simulink model "sf_clutch"  (R2025b)
settings: Solver=ode45  StartTime=0.0  StopTime=10  RelTol=1e-6  AbsTol=1e-7
model workspace (MATLAB code in the model file):
  | % Load initial conditions and other information
  | 
  | load sf_clutch_data.mat;
undefined symbols (not defined in the file or in its folder): be, bv, Ie, Iv, muk, mus, R
Description:
  | Building a Clutch Lock-Up Model
  | 
  | This example shows how to use Simulink(R) to model and simulate a
  | rotating clutch system. Although modeling a clutch system is difficult
  | because of topological changes in the system dynamics during lockup, this
  | example shows how Simulinks enabled subsystems feature easily handles
  | such problems. We illustrate how to employ important Simulink modeling
  | concepts in the creation of the clutch simulation. Designers can apply
  | these concepts to many models with strong discontinuities and constraints
  | that may change dynamically.
  | 
  | In the example, we use enabled subsystems to build the clutch
  | model. Two enabled subsystems model the clutch dynamics in either the
  | locked or unlocked position. After running the simulation, a GUI opens.
  | Checking any of the boxes on the GUI produces a plot of any of the
  | selected variables (versus time).
settings Model: ExtModeTrigMode=oneshot  ExtModeArmWhenConnect=off  ExtModeAutoUpdateStatusClock=off  Creator=The MathWorks, Inc.  LastModifiedBy=The MathWorks, Inc.
settings SolverCC: AutoScaleAbsTol=off  ZeroCrossAlgorithm=Adaptive  AlgebraicLoopSolver=TrustRegion  MaxZcPerStep=1.0
settings DataIOCC: ExternalInput=[]  InitialState=[]  SaveFormat=Array  SaveState=on  DSMLogging=off  ReturnWorkspaceOutputs=off  StateSaveName=x  TimeSaveName=t  OutputSaveName=y  SignalLoggingName=sf_clutch_signals
settings OptimizationCC: BlockReduction=off  ReuseModelBlockBuffer=off  ExpressionDepthLimit=2147483647.0  InitFltsAndDblsToZero=on  LifeSpan=inf  BufferReusableBoundary=off
settings DebuggingCC: SaveWithParameterizedLinksMsg=none  SignalResolutionControl=TryResolveAllWithWarning  MultiTaskDSMMsg=warning  MultiTaskCondExecSysMsg=none  SigSpecEnsureSampleTimeMsg=none  IntegerOverflowMsg=none  FcnCallInpInsideContextMsg=warning  UnconnectedInputMsg=warning  UnconnectedOutputMsg=warning  UnconnectedLineMsg=warning  BusObjectLabelMismatch=none  AllowSymbolicDim=off  StateNameClashWarn=warning  SFUnexpectedBacktrackingDiag=warning  SFNoUnconditionalDefaultTransitionDiag=warning  SFExecutionAtInitializationDiag=none  IntegerSaturationMsg=none  ArithmeticOperatorsInVariantConditions=warning
settings HardwareCC: ProdBitPerPointer=32.0  ProdBitPerSizeT=32.0  ProdBitPerPtrDiffT=32.0  ProdLargestAtomicFloat=None  ProdIntDivRoundTo=Undefined  ProdEndianess=Unspecified  ProdWordSize=32.0  ProdHWDeviceType=32-bit Generic
settings ModelReferenceCC: EnableRefExpFcnMdlSchedulingChecks=on  PropagateSignalLabelsOutOfModel=off
settings SFSimCC: SimUseLocalCustomCode=off  CustomCodeUndefinedFunction=UseInterfaceOnly
settings RTWCC: RTWUseLocalCustomCode=off  GPUComputeCapability=3.5  DLArmComputeVersion=19.05
settings CodeAppCC: StateflowObjectComments=on
settings GRTTargetCC: TargetFcnLib=ansi_tfl_tmw.mat  TargetLangStandard=C89/C90 (ANSI)  CombineOutputUpdateFcns=off  GRTInterface=on
settings ConfigComp: CovMetricSettings=d  CovSaveCumulativeToWorkspaceVar=on  CovSaveSingleToWorkspaceVar=on  CovExternalEMLEnable=off

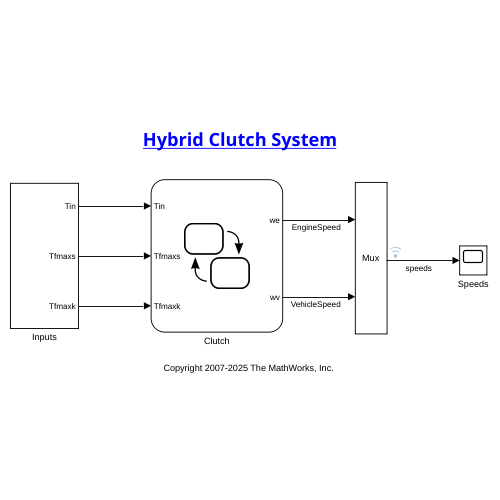
[thumbnail: Simulink's stored preview of the top-level diagram]
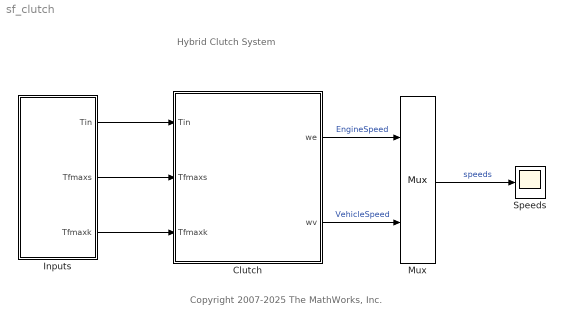
== system sf_clutch ==
  note: Copyright 2007-2025 The MathWorks, Inc.
  note: Hybrid Clutch System
  Clutch : Stateflow chart  TreatAsAtomicUnit=on
  Inputs : Subsystem
  Mux : Mux  Inputs=2
  Speeds : Scope
      settings: TimeSpan=10  ActiveDisplayYMinimum=-0.08933  ActiveDisplayYMaximum=0.80399
  wires:
  Clutch/1(we) -> Mux/1  "EngineSpeed"
  Clutch/2(wv) -> Mux/2  "VehicleSpeed"
  Mux/1 -> Speeds/1  "speeds"
  Inputs/1(Tin) -> Clutch/1(Tin)
  Inputs/2(Tfmaxs) -> Clutch/2(Tfmaxs)
  Inputs/3(Tfmaxk) -> Clutch/3(Tfmaxk)

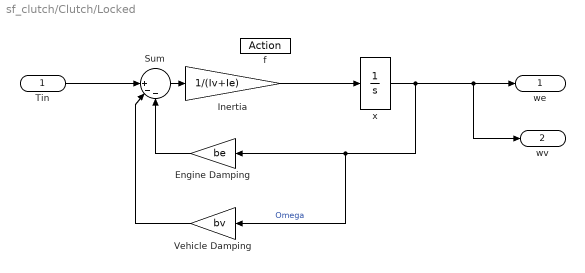
== system sf_clutch/Clutch/Locked ==
  Tin : Inport
  f : ActionPort
      settings: CopyFcn=Stateflow.SLINSF.SimulinkMan.removeBlockPreDeleteFcn  PreDeleteFcn=Stateflow.SLINSF.SimulinkMan.unsafePredeleteFcn
  Engine Damping : Gain  Gain=be  SaturateOnIntegerOverflow=on  OutDataTypeStr=Inherit: Same as input  ParamDataTypeStr=Inherit: Same as input
  Inertia : Gain  Gain=1/(Iv+Ie)  SaturateOnIntegerOverflow=on  OutDataTypeStr=Inherit: Same as input  ParamDataTypeStr=Inherit: Same as input
  Sum : Sum  Inputs=||+--  InputSameDT=on  SaturateOnIntegerOverflow=on  OutDataTypeStr=Inherit: Same as first input
  Vehicle Damping : Gain  Gain=bv  SaturateOnIntegerOverflow=on  OutDataTypeStr=Inherit: Same as input  ParamDataTypeStr=Inherit: Same as input
  x : Integrator  ContinuousStateAttributes='w'
  we : Outport  VectorParamsAs1DForOutWhenUnconnected=off
  wv : Outport  Port=2  VectorParamsAs1DForOutWhenUnconnected=off
  wires:
  Sum/1 -> Inertia/1
  Tin/1 -> Sum/1
  x/1 -> wv/1, we/1, Engine Damping/1, Vehicle Damping/1  "Omega"
  Engine Damping/1 -> Sum/3
  Inertia/1 -> x/1
  Vehicle Damping/1 -> Sum/2

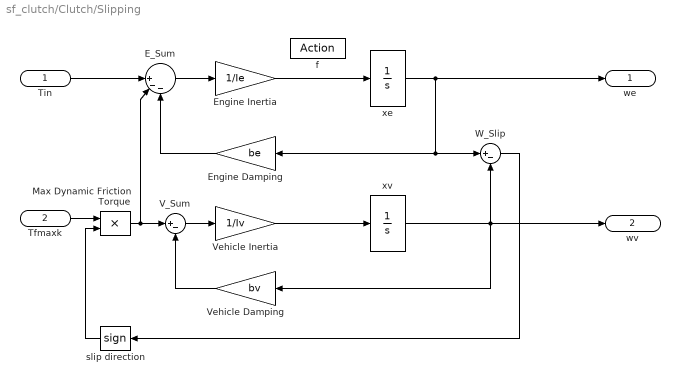
== system sf_clutch/Clutch/Slipping ==
  Tin : Inport
  Tfmaxk : Inport  Port=2
  f : ActionPort
      settings: CopyFcn=Stateflow.SLINSF.SimulinkMan.removeBlockPreDeleteFcn  PreDeleteFcn=Stateflow.SLINSF.SimulinkMan.unsafePredeleteFcn
  E_Sum : Sum  Inputs=||+--  InputSameDT=on  SaturateOnIntegerOverflow=on  OutDataTypeStr=Inherit: Same as first input
  Engine Damping : Gain  Gain=be  SaturateOnIntegerOverflow=on  OutDataTypeStr=Inherit: Same as input  ParamDataTypeStr=Inherit: Same as input
  Engine Inertia : Gain  Gain=1/Ie  SaturateOnIntegerOverflow=on  OutDataTypeStr=Inherit: Same as input  ParamDataTypeStr=Inherit: Same as input
  Max Dynamic Friction Torque : Product  InputSameDT=on  RndMeth=Zero  SaturateOnIntegerOverflow=on  OutDataTypeStr=Inherit: Same as first input
  V_Sum : Sum  Inputs=|+-  InputSameDT=on  SaturateOnIntegerOverflow=on  OutDataTypeStr=Inherit: Same as first input
  Vehicle Damping : Gain  Gain=bv  SaturateOnIntegerOverflow=on  OutDataTypeStr=Inherit: Same as input  ParamDataTypeStr=Inherit: Same as input
  Vehicle Inertia : Gain  Gain=1/Iv  SaturateOnIntegerOverflow=on  OutDataTypeStr=Inherit: Same as input  ParamDataTypeStr=Inherit: Same as input
  W_Slip : Sum  Inputs=|+-  InputSameDT=on  SaturateOnIntegerOverflow=on  OutDataTypeStr=Inherit: Same as first input
  slip direction : Signum
  xe : Integrator  ContinuousStateAttributes='we'
  xv : Integrator  ContinuousStateAttributes='wv'
  we : Outport  VectorParamsAs1DForOutWhenUnconnected=off
  wv : Outport  Port=2  VectorParamsAs1DForOutWhenUnconnected=off
  wires:
  V_Sum/1 -> Vehicle Inertia/1
  Vehicle Damping/1 -> V_Sum/2
  Max Dynamic Friction Torque/1 -> V_Sum/1, E_Sum/2
  Tfmaxk/1 -> Max Dynamic Friction Torque/1
  slip direction/1 -> Max Dynamic Friction Torque/2
  W_Slip/1 -> slip direction/1
  Engine Inertia/1 -> xe/1
  E_Sum/1 -> Engine Inertia/1
  Engine Damping/1 -> E_Sum/3
  Tin/1 -> E_Sum/1
  Vehicle Inertia/1 -> xv/1
  xe/1 -> we/1, Engine Damping/1, W_Slip/1
  xv/1 -> wv/1, Vehicle Damping/1, W_Slip/2

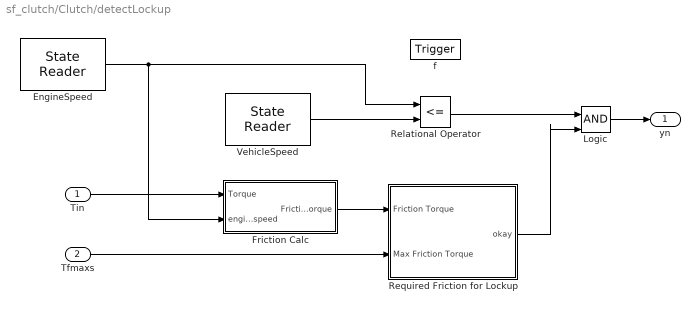
== system sf_clutch/Clutch/detectLockup ==
  Tin : Inport
  Tfmaxs : Inport  Port=2
  f : TriggerPort  TriggerType=function-call  VariantControl=Variant
      settings: CopyFcn=Stateflow.SLINSF.SimulinkMan.removeBlockPreDeleteFcn  PreDeleteFcn=Stateflow.SLINSF.SimulinkMan.unsafePredeleteFcn
  EngineSpeed : StateReader  StateOwnerBlock=../../Slipping/xe  StateName=we
  Friction Calc : Subsystem
  Logic : Logic  IconShape=distinctive  OutDataTypeStr=boolean
  Relational Operator : RelationalOperator  Operator=<=  OutDataTypeStr=boolean  InputSameDT=off
  Required Friction for Lockup : Subsystem
  VehicleSpeed : StateReader  StateOwnerBlock=../../Slipping/xv  StateName=wv
  yn : Outport  VectorParamsAs1DForOutWhenUnconnected=off
  wires:
  Friction Calc/1(Friction Torque) -> Required Friction for Lockup/1(Friction Torque)
  Tfmaxs/1 -> Required Friction for Lockup/2(Max Friction Torque)
  Relational Operator/1 -> Logic/1
  Required Friction for Lockup/1(okay) -> Logic/2
  EngineSpeed/1 -> Friction Calc/2(engine speed), Relational Operator/1
  VehicleSpeed/1 -> Relational Operator/2
  Tin/1 -> Friction Calc/1(Torque)
  Logic/1 -> yn/1

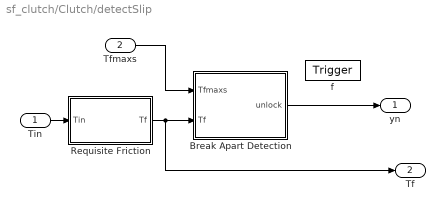
== system sf_clutch/Clutch/detectSlip ==
  Tin : Inport
  Tfmaxs : Inport  Port=2
  f : TriggerPort  TriggerType=function-call  VariantControl=Variant
      settings: CopyFcn=Stateflow.SLINSF.SimulinkMan.removeBlockPreDeleteFcn  PreDeleteFcn=Stateflow.SLINSF.SimulinkMan.unsafePredeleteFcn
  Break Apart Detection : Subsystem
  Requisite Friction : Subsystem
  yn : Outport  VectorParamsAs1DForOutWhenUnconnected=off
  Tf : Outport  Port=2  VectorParamsAs1DForOutWhenUnconnected=off
  wires:
  Tfmaxs/1 -> Break Apart Detection/1(Tfmaxs)
  Requisite Friction/1(Tf) -> Tf/1, Break Apart Detection/2(Tf)
  Break Apart Detection/1(unlock) -> yn/1
  Tin/1 -> Requisite Friction/1(Tin)

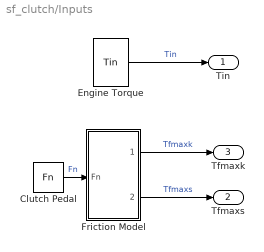
== system sf_clutch/Inputs ==
  Clutch Pedal : FromWorkspace  VariableName=Fn  ZeroCross=off
  Engine Torque : FromWorkspace  VariableName=Tin  ZeroCross=off
  Friction Model : Subsystem
  Tin : Outport  VectorParamsAs1DForOutWhenUnconnected=off
  Tfmaxs : Outport  Port=2  VectorParamsAs1DForOutWhenUnconnected=off
  Tfmaxk : Outport  Port=3  VectorParamsAs1DForOutWhenUnconnected=off
  wires:
  Clutch Pedal/1 -> Friction Model/1(Fn)  "Fn"
  Engine Torque/1 -> Tin/1  "Tin"
  Friction Model/1(Tfmaxk) -> Tfmaxk/1  "Tfmaxk"
  Friction Model/2(Tfmaxs) -> Tfmaxs/1  "Tfmaxs"

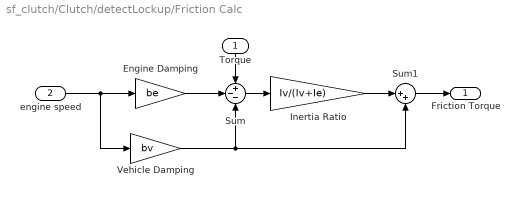
== system sf_clutch/Clutch/detectLockup/Friction Calc ==
  Torque : Inport
  engine speed : Inport  Port=2
  Engine Damping : Gain  Gain=be  SaturateOnIntegerOverflow=on  OutDataTypeStr=Inherit: Same as input  ParamDataTypeStr=Inherit: Same as input
  Inertia Ratio : Gain  Gain=Iv/(Iv+Ie)  SaturateOnIntegerOverflow=on  OutDataTypeStr=Inherit: Same as input  ParamDataTypeStr=Inherit: Same as input
  Sum : Sum  Inputs=+--  InputSameDT=on  SaturateOnIntegerOverflow=on  OutDataTypeStr=Inherit: Same as first input
  Sum1 : Sum  Inputs=|++  InputSameDT=on  SaturateOnIntegerOverflow=on  OutDataTypeStr=Inherit: Same as first input
  Vehicle Damping : Gain  Gain=bv  SaturateOnIntegerOverflow=on  OutDataTypeStr=Inherit: Same as input  ParamDataTypeStr=Inherit: Same as input
  Friction Torque : Outport  InitialOutput=0  VectorParamsAs1DForOutWhenUnconnected=off
  wires:
  engine speed/1 -> Engine Damping/1, Vehicle Damping/1
  Vehicle Damping/1 -> Sum1/2, Sum/3
  Engine Damping/1 -> Sum/2
  Sum/1 -> Inertia Ratio/1
  Torque/1 -> Sum/1
  Inertia Ratio/1 -> Sum1/1
  Sum1/1 -> Friction Torque/1

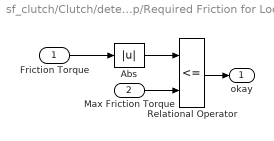
== system sf_clutch/Clutch/detectLockup/Required Friction for Lockup ==
  Friction Torque : Inport
  Max Friction Torque : Inport  Port=2
  Abs : Abs
  Relational Operator : RelationalOperator  Operator=<=  OutDataTypeStr=boolean
  okay : Outport  InitialOutput=0  VectorParamsAs1DForOutWhenUnconnected=off
  wires:
  Friction Torque/1 -> Abs/1
  Relational Operator/1 -> okay/1
  Abs/1 -> Relational Operator/1
  Max Friction Torque/1 -> Relational Operator/2

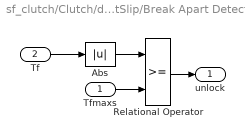
== system sf_clutch/Clutch/detectSlip/Break Apart Detection ==
  Tfmaxs : Inport
  Tf : Inport  Port=2
  Abs : Abs
  Relational Operator : RelationalOperator  OutDataTypeStr=boolean
  unlock : Outport  InitialOutput=0  VectorParamsAs1DForOutWhenUnconnected=off
  wires:
  Tf/1 -> Abs/1
  Relational Operator/1 -> unlock/1
  Abs/1 -> Relational Operator/1
  Tfmaxs/1 -> Relational Operator/2

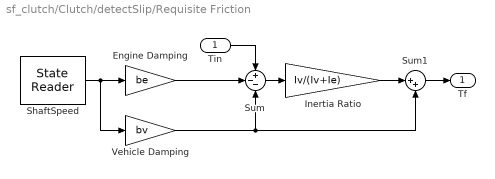
== system sf_clutch/Clutch/detectSlip/Requisite Friction ==
  Tin : Inport
  Engine Damping : Gain  Gain=be  SaturateOnIntegerOverflow=on  OutDataTypeStr=Inherit: Same as input  ParamDataTypeStr=Inherit: Same as input
  Inertia Ratio : Gain  Gain=Iv/(Iv+Ie)  SaturateOnIntegerOverflow=on  OutDataTypeStr=Inherit: Same as input  ParamDataTypeStr=Inherit: Same as input
  ShaftSpeed : StateReader  StateOwnerBlock=../../../Locked/x  StateName=w
  Sum : Sum  Inputs=+--  InputSameDT=on  SaturateOnIntegerOverflow=on  OutDataTypeStr=Inherit: Same as first input
  Sum1 : Sum  Inputs=|++  InputSameDT=on  SaturateOnIntegerOverflow=on  OutDataTypeStr=Inherit: Same as first input
  Vehicle Damping : Gain  Gain=bv  SaturateOnIntegerOverflow=on  OutDataTypeStr=Inherit: Same as input  ParamDataTypeStr=Inherit: Same as input
  Tf : Outport  InitialOutput=0  VectorParamsAs1DForOutWhenUnconnected=off
  wires:
  ShaftSpeed/1 -> Vehicle Damping/1, Engine Damping/1
  Engine Damping/1 -> Sum/2
  Vehicle Damping/1 -> Sum/3, Sum1/2
  Sum/1 -> Inertia Ratio/1
  Tin/1 -> Sum/1
  Inertia Ratio/1 -> Sum1/1
  Sum1/1 -> Tf/1

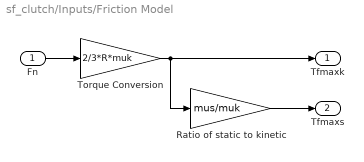
== system sf_clutch/Inputs/Friction Model ==
  Fn : Inport
  Ratio of static to kinetic : Gain  Gain=mus/muk  SaturateOnIntegerOverflow=on  OutDataTypeStr=Inherit: Same as input  ParamDataTypeStr=Inherit: Same as input
  Torque Conversion : Gain  Gain=2/3*R*muk  SaturateOnIntegerOverflow=on  OutDataTypeStr=Inherit: Same as input  ParamDataTypeStr=Inherit: Same as input
  Tfmaxk : Outport  InitialOutput=0  VectorParamsAs1DForOutWhenUnconnected=off
  Tfmaxs : Outport  Port=2  InitialOutput=0  VectorParamsAs1DForOutWhenUnconnected=off
  wires:
  Torque Conversion/1 -> Tfmaxk/1, Ratio of static to kinetic/1
  Fn/1 -> Torque Conversion/1
  Ratio of static to kinetic/1 -> Tfmaxs/1

== stateflow chart sf_clutch/Clutch ==
  settings: updateMethod=CONTINUOUS
  state Slipping
  state yn = detectLockup(Tin,Tfmaxs) [function]
  state [yn,Tf] = detectSlip(Tin,Tfmaxs) [function]
  state Locked
  (default) -> Slipping
  Slipping -> Locked : [detectLockup(Tin, Tfmaxs)]
      | {Locked.w = Slipping.we;}
  Locked -> Slipping : [detectSlip(Tin,Tfmaxs)]
      | {
      | Slipping.we = Locked.w;
      | Slipping.wv = Locked.w;
      | }
  data: sf_internal_action_state_placeholder_data local double size=1 =0; we local; wv local; yn function_output; Tin function_input; Tfmaxs function_input; yn function_output; Tin function_input; Tfmaxs function_input; Tf function_output; sf_internal_action_state_placeholder_data local double size=1 =0; w local; we output double; wv output double; Tin input double; Tfmaxs input double; Tfmaxk input double
